simulink model "system_simulation_FC"  (R2025b)
settings: Solver=FixedStepAuto  StartTime=0.0  StopTime=12  FixedStep=Ts/10  RelTol=1e-3
model workspace (MAT data in the model file):
  aprbs_seed = 10
  u_hover = [0.385; 0.385; 0.385; 0.385]
values from neighbouring files (symbols this model uses):
  horizon_N = 20    [main_simulation.m]    (also in random_init.m)
  Ts = 0.05    [generate_commande_preview.m]    (also in random_init.m)
libraries: slpidlib x4
settings Model: Creator=Max  LastModifiedBy=cs_fondation
settings SolverCC: AlgebraicLoopSolver=TrustRegion
settings DebuggingCC: UnconnectedInputMsg=warning  UnconnectedOutputMsg=warning  UnconnectedLineMsg=warning
settings ModelReferenceCC: EnableRefExpFcnMdlSchedulingChecks=on
settings RTWCC: GPUComputeCapability=3.5

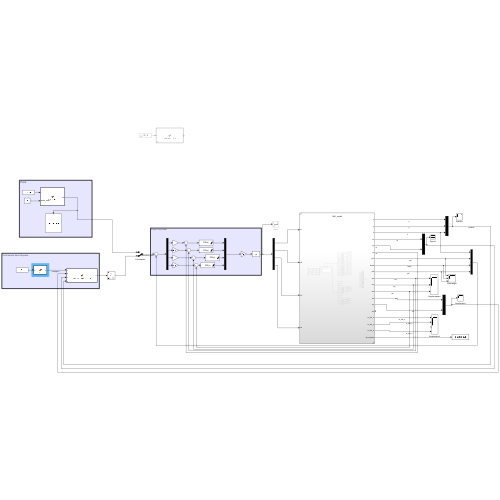
[thumbnail: Simulink's stored preview of the top-level diagram]
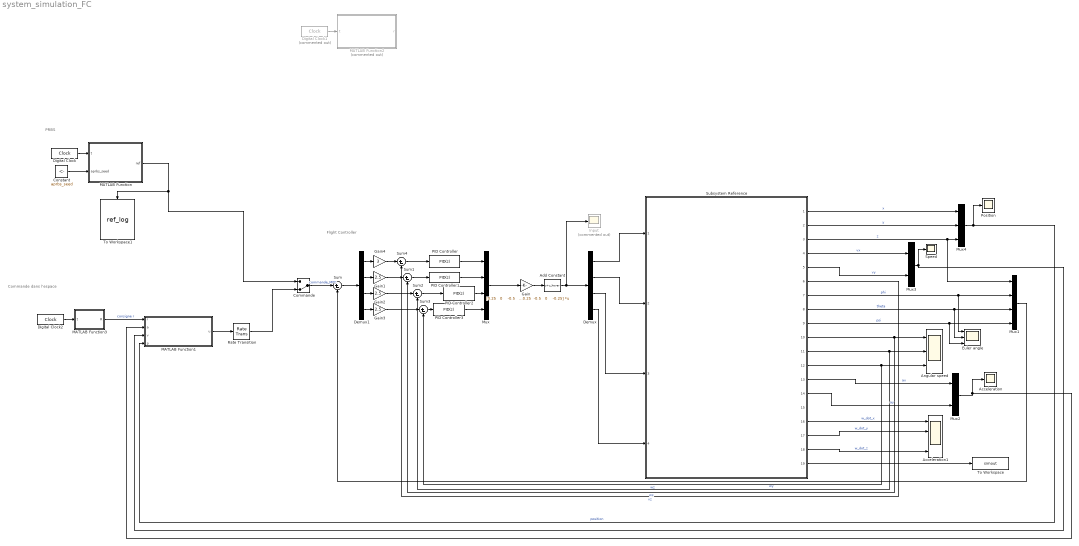
== system system_simulation_FC ==
  note: Commande dans l'espace
  note: Flight Controller
  note: PRBS
  Acceleration : Scope
      settings: ActiveDisplayYMinimum=-12.148465350315172  ActiveDisplayYMaximum=11.235939995916615
  Acceleration1 : Scope  NumInputPorts=4
      settings: ActiveDisplayYMinimum=-40.918121722117149  ActiveDisplayYMaximum=44.001627281329164  DataLoggingVariableName=ScopeData2
  Add Constant : Bias  Bias=u_hover  SaturateOnIntegerOverflow=off
  Angular speed : Scope  NumInputPorts=3
      settings: ActiveDisplayYMinimum=-1  ActiveDisplayYMaximum=1  DataLoggingVariableName=ScopeData3
  Commande : ManualSwitch  CurrentSetting=0
  Constant : Constant  Value=aprbs_seed
  Demux : Demux
  Demux1 : Demux
  Digital Clock : DigitalClock  SampleTime=Ts
  Digital Clock1 : DigitalClock  Commented=on  SampleTime=Ts
  Digital Clock2 : DigitalClock  SampleTime=Ts
  Euler angle : Scope  NumInputPorts=3
      settings: ActiveDisplayYMinimum=-0.25591734670833521  ActiveDisplayYMaximum=0.42163771962698082  DataLoggingVariableName=ScopeData4
  Gain : Gain  Gain=|  Multiplication=Matrix(K*u)
      | [0.25   0    -0.5   0.25;
      |  0.25   0.5   0    -0.25;
      |  0.25   0     0.5   0.25;
      |  0.25  -0.5   0    -0.25]
  Gain1 : Gain  Gain=2.5
  Gain2 : Gain  Gain=2.5
  Gain3 : Gain  Gain=2.5
  Gain4 : Gain  Gain=3
  Input : Scope  Commented=on
      settings: ActiveDisplayYMinimum=-1.25  ActiveDisplayYMaximum=1.25  DataLoggingVariableName=ScopeData5
  MATLAB Function : MATLAB Function  TreatAsAtomicUnit=on
  MATLAB Function1 : MATLAB Function  TreatAsAtomicUnit=on
  MATLAB Function2 : MATLAB Function  Commented=on  TreatAsAtomicUnit=on
  MATLAB Function3 : MATLAB Function  TreatAsAtomicUnit=on
  Mux : Mux
  Mux1 : Mux
  Mux2 : Mux  Inputs=2
  Mux3 : Mux  Inputs=2
  Mux4 : Mux  Inputs=3
  PID Controller : slpidlib/PID Controller  Controller=PID  Form=Parallel  TimeDomain=Discrete-time  UseExternalTs=off  SampleTime=0.005  IntegratorMethod=Forward Euler  FilterMethod=Forward Euler  ControllerParametersSource=internal  P=2.08  I=0.2  UseKiTs=off  D=0.42  UseExternalDerivativeSource=off  N=100  UseFilter=on  TunerSelectOption=Transfer Function Based (PID Tuner App)  InitialConditionSource=internal  InitialConditionForIntegrator=0  InitialConditionForFilter=0  DifferentiatorICPrevScaledInput=0  ExternalReset=none  TrackingMode=off  Kt=1  LimitOutput=on  SatLimitsSource=internal  UpperSaturationLimit=4*(1 - max(u_hover))  LowerSaturationLimit=-4*min(u_hover)  LinearizeAsGain=off  AntiWindupMode=clamping  Kb=1  LimitIntegrator=off  UpperIntegratorSaturationLimit=inf  LowerIntegratorSaturationLimit=-inf  POutMin=[]  POutMax=[]  IOutMin=[]  IOutMax=[]  DOutMin=[]  DOutMax=[]  NOutMin=[]  NOutMax=[]  SumOutMin=[]  SumOutMax=[]  SaturationOutMin=[]  SaturationOutMax=[]  PParamMin=[]  PParamMax=[]  IParamMin=[]  IParamMax=[]  DParamMin=[]  DParamMax=[]  NParamMin=[]  NParamMax=[]  KbParamMin=[]  KbParamMax=[]  KtParamMin=[]  KtParamMax=[]  KbOutMin=[]  KbOutMax=[]  KtOutMin=[]  KtOutMax=[]  IntegratorOutMin=[]  IntegratorOutMax=[]  FilterOutMin=[]  FilterOutMax=[]  SumI1OutMin=[]  SumI1OutMax=[]  SumI2OutMin=[]  SumI2OutMax=[]  SumI3OutMin=[]  SumI3OutMax=[]  SumI4OutMin=[]  SumI4OutMax=[]  SumDOutMin=[]  SumDOutMax=[]  DifferentiatorOutMin=[]  DifferentiatorOutMax=[]  FilterDiffOutCoefMin=[]  FilterDiffOutCoefMax=[]  ReciprocalOutMin=[]  ReciprocalOutMax=[]  SumDenOutMin=[]  SumDenOutMax=[]  SumNumOutMin=[]  SumNumOutMax=[]  DivideOutMin=[]  DivideOutMax=[]  UdiffTsProdOutMin=[]  UdiffTsProdOutMax=[]  NTsProdOutMin=[]  NTsProdOutMax=[]  UintegralTsProdOutMin=[]  UintegralTsProdOutMax=[]  UngainTsProdOutMin=[]  UngainTsProdOutMax=[]  ClampingZeroOutDataTypeStr=Inherit: Inherit via back propagation  ClampingZeroOutMin=[]  ClampingZeroOutMax=[]  FilterDenConstantOutDataTypeStr=Inherit: Inherit via back propagation  FilterDenConstantOutMin=[]  FilterDenConstantOutMax=[]  PCopyOutDataTypeStr=Inherit: Inherit via back propagation  PCopyOutMin=[]  PCopyOutMax=[]  NCopyOutDataTypeStr=Inherit: Inherit via back propagation  NCopyOutMin=[]  NCopyOutMax=[]  IntegratorContinuousStateAttributes=''  IntegratorStateMustResolveToSignalObject=off  IntegratorRTWStateStorageClass=Auto  FilterContinuousStateAttributes=''  FilterStateMustResolveToSignalObject=off  FilterRTWStateStorageClass=Auto  ParallelPVariant=InternalParameters  IdealPVariant=Disabled  IVariant=InternalParameters  DVariant=InternalParameters  IntegratorVariant=Discrete  SatVariant=Enabled  AWVariant=DiscClampingParallel  PCopyVariant=Disabled  TRVariant=Disabled  FdbkBlocksVariant=Forward  IdealPFdbkVariant=Disabled  SatFdbkVariant=Disabled  DerivativeFilterVariant=ForwardEulerFilter  NVariant=InternalParameters  NCopyVariant=Disabled  FilterICVariant=InternalICsFilter  IntegratorICVariant=InternalICs  ExternalResetVariant=Disabled  TRSumVariant=Passthrough  SumFdbkVariant=Disabled  SumVariant=Sum_PID  TsampFilterVariant=InternalTs  TsampNgainVariant=Passthrough  TsampIntegralVariant=Disabled_SignalSpec  ExternalSaturationOutDataTypeStr=Inherit: Same as second input  DerivativeSourceVariant=ErrorSignal  PreIntVariant=InternalPreInt
  PID Controller1 : slpidlib/PID Controller  Controller=PID  Form=Parallel  TimeDomain=Discrete-time  UseExternalTs=off  SampleTime=0.005  IntegratorMethod=Forward Euler  FilterMethod=Forward Euler  ControllerParametersSource=internal  P=0.125  I=0.05  UseKiTs=off  D=0.025  UseExternalDerivativeSource=off  N=100  UseFilter=on  TunerSelectOption=Transfer Function Based (PID Tuner App)  InitialConditionSource=internal  InitialConditionForIntegrator=0  InitialConditionForFilter=0  DifferentiatorICPrevScaledInput=0  ExternalReset=none  TrackingMode=off  Kt=1  LimitOutput=on  SatLimitsSource=internal  UpperSaturationLimit=2*min([u_hover(:); 1 - u_hover(:)])  LowerSaturationLimit=-2*min([u_hover(:); 1 - u_hover(:)])  LinearizeAsGain=on  AntiWindupMode=clamping  Kb=1  LimitIntegrator=off  UpperIntegratorSaturationLimit=inf  LowerIntegratorSaturationLimit=-inf  POutMin=[]  POutMax=[]  IOutMin=[]  IOutMax=[]  DOutMin=[]  DOutMax=[]  NOutMin=[]  NOutMax=[]  SumOutMin=[]  SumOutMax=[]  SaturationOutMin=[]  SaturationOutMax=[]  PParamMin=[]  PParamMax=[]  IParamMin=[]  IParamMax=[]  DParamMin=[]  DParamMax=[]  NParamMin=[]  NParamMax=[]  KbParamMin=[]  KbParamMax=[]  KtParamMin=[]  KtParamMax=[]  KbOutMin=[]  KbOutMax=[]  KtOutMin=[]  KtOutMax=[]  IntegratorOutMin=[]  IntegratorOutMax=[]  FilterOutMin=[]  FilterOutMax=[]  SumI1OutMin=[]  SumI1OutMax=[]  SumI2OutMin=[]  SumI2OutMax=[]  SumI3OutMin=[]  SumI3OutMax=[]  SumI4OutMin=[]  SumI4OutMax=[]  SumDOutMin=[]  SumDOutMax=[]  DifferentiatorOutMin=[]  DifferentiatorOutMax=[]  FilterDiffOutCoefMin=[]  FilterDiffOutCoefMax=[]  ReciprocalOutMin=[]  ReciprocalOutMax=[]  SumDenOutMin=[]  SumDenOutMax=[]  SumNumOutMin=[]  SumNumOutMax=[]  DivideOutMin=[]  DivideOutMax=[]  UdiffTsProdOutMin=[]  UdiffTsProdOutMax=[]  NTsProdOutMin=[]  NTsProdOutMax=[]  UintegralTsProdOutMin=[]  UintegralTsProdOutMax=[]  UngainTsProdOutMin=[]  UngainTsProdOutMax=[]  ClampingZeroOutDataTypeStr=Inherit: Inherit via back propagation  ClampingZeroOutMin=[]  ClampingZeroOutMax=[]  FilterDenConstantOutDataTypeStr=Inherit: Inherit via back propagation  FilterDenConstantOutMin=[]  FilterDenConstantOutMax=[]  PCopyOutDataTypeStr=Inherit: Inherit via back propagation  PCopyOutMin=[]  PCopyOutMax=[]  NCopyOutDataTypeStr=Inherit: Inherit via back propagation  NCopyOutMin=[]  NCopyOutMax=[]  IntegratorContinuousStateAttributes=''  IntegratorStateMustResolveToSignalObject=off  IntegratorRTWStateStorageClass=Auto  FilterContinuousStateAttributes=''  FilterStateMustResolveToSignalObject=off  FilterRTWStateStorageClass=Auto  ParallelPVariant=InternalParameters  IdealPVariant=Disabled  IVariant=InternalParameters  DVariant=InternalParameters  IntegratorVariant=Discrete  SatVariant=Enabled  AWVariant=DiscClampingParallel  PCopyVariant=Disabled  TRVariant=Disabled  FdbkBlocksVariant=Forward  IdealPFdbkVariant=Disabled  SatFdbkVariant=Disabled  DerivativeFilterVariant=ForwardEulerFilter  NVariant=InternalParameters  NCopyVariant=Disabled  FilterICVariant=InternalICsFilter  IntegratorICVariant=InternalICs  ExternalResetVariant=Disabled  TRSumVariant=Passthrough  SumFdbkVariant=Disabled  SumVariant=Sum_PID  TsampFilterVariant=InternalTs  TsampNgainVariant=Passthrough  TsampIntegralVariant=Disabled_SignalSpec  ExternalSaturationOutDataTypeStr=Inherit: Same as second input  DerivativeSourceVariant=ErrorSignal  PreIntVariant=InternalPreInt
  PID Controller2 : slpidlib/PID Controller  Controller=PID  Form=Parallel  TimeDomain=Discrete-time  UseExternalTs=off  SampleTime=0.005  IntegratorMethod=Forward Euler  FilterMethod=Forward Euler  ControllerParametersSource=internal  P=0.125  I=0.05  UseKiTs=off  D=0.025  UseExternalDerivativeSource=off  N=100  UseFilter=on  TunerSelectOption=Transfer Function Based (PID Tuner App)  InitialConditionSource=internal  InitialConditionForIntegrator=0  InitialConditionForFilter=0  DifferentiatorICPrevScaledInput=0  ExternalReset=none  TrackingMode=off  Kt=1  LimitOutput=on  SatLimitsSource=internal  UpperSaturationLimit=2*min([u_hover(:); 1 - u_hover(:)])  LowerSaturationLimit=-2*min([u_hover(:); 1 - u_hover(:)])  LinearizeAsGain=on  AntiWindupMode=clamping  Kb=1  LimitIntegrator=off  UpperIntegratorSaturationLimit=inf  LowerIntegratorSaturationLimit=-inf  POutMin=[]  POutMax=[]  IOutMin=[]  IOutMax=[]  DOutMin=[]  DOutMax=[]  NOutMin=[]  NOutMax=[]  SumOutMin=[]  SumOutMax=[]  SaturationOutMin=[]  SaturationOutMax=[]  PParamMin=[]  PParamMax=[]  IParamMin=[]  IParamMax=[]  DParamMin=[]  DParamMax=[]  NParamMin=[]  NParamMax=[]  KbParamMin=[]  KbParamMax=[]  KtParamMin=[]  KtParamMax=[]  KbOutMin=[]  KbOutMax=[]  KtOutMin=[]  KtOutMax=[]  IntegratorOutMin=[]  IntegratorOutMax=[]  FilterOutMin=[]  FilterOutMax=[]  SumI1OutMin=[]  SumI1OutMax=[]  SumI2OutMin=[]  SumI2OutMax=[]  SumI3OutMin=[]  SumI3OutMax=[]  SumI4OutMin=[]  SumI4OutMax=[]  SumDOutMin=[]  SumDOutMax=[]  DifferentiatorOutMin=[]  DifferentiatorOutMax=[]  FilterDiffOutCoefMin=[]  FilterDiffOutCoefMax=[]  ReciprocalOutMin=[]  ReciprocalOutMax=[]  SumDenOutMin=[]  SumDenOutMax=[]  SumNumOutMin=[]  SumNumOutMax=[]  DivideOutMin=[]  DivideOutMax=[]  UdiffTsProdOutMin=[]  UdiffTsProdOutMax=[]  NTsProdOutMin=[]  NTsProdOutMax=[]  UintegralTsProdOutMin=[]  UintegralTsProdOutMax=[]  UngainTsProdOutMin=[]  UngainTsProdOutMax=[]  ClampingZeroOutDataTypeStr=Inherit: Inherit via back propagation  ClampingZeroOutMin=[]  ClampingZeroOutMax=[]  FilterDenConstantOutDataTypeStr=Inherit: Inherit via back propagation  FilterDenConstantOutMin=[]  FilterDenConstantOutMax=[]  PCopyOutDataTypeStr=Inherit: Inherit via back propagation  PCopyOutMin=[]  PCopyOutMax=[]  NCopyOutDataTypeStr=Inherit: Inherit via back propagation  NCopyOutMin=[]  NCopyOutMax=[]  IntegratorContinuousStateAttributes=''  IntegratorStateMustResolveToSignalObject=off  IntegratorRTWStateStorageClass=Auto  FilterContinuousStateAttributes=''  FilterStateMustResolveToSignalObject=off  FilterRTWStateStorageClass=Auto  ParallelPVariant=InternalParameters  IdealPVariant=Disabled  IVariant=InternalParameters  DVariant=InternalParameters  IntegratorVariant=Discrete  SatVariant=Enabled  AWVariant=DiscClampingParallel  PCopyVariant=Disabled  TRVariant=Disabled  FdbkBlocksVariant=Forward  IdealPFdbkVariant=Disabled  SatFdbkVariant=Disabled  DerivativeFilterVariant=ForwardEulerFilter  NVariant=InternalParameters  NCopyVariant=Disabled  FilterICVariant=InternalICsFilter  IntegratorICVariant=InternalICs  ExternalResetVariant=Disabled  TRSumVariant=Passthrough  SumFdbkVariant=Disabled  SumVariant=Sum_PID  TsampFilterVariant=InternalTs  TsampNgainVariant=Passthrough  TsampIntegralVariant=Disabled_SignalSpec  ExternalSaturationOutDataTypeStr=Inherit: Same as second input  DerivativeSourceVariant=ErrorSignal  PreIntVariant=InternalPreInt
  PID Controller3 : slpidlib/PID Controller  Controller=PID  Form=Parallel  TimeDomain=Discrete-time  UseExternalTs=off  SampleTime=0.005  IntegratorMethod=Forward Euler  FilterMethod=Forward Euler  ControllerParametersSource=internal  P=0.23  I=0.093  UseKiTs=off  D=0.047  UseExternalDerivativeSource=off  N=100  UseFilter=on  TunerSelectOption=Transfer Function Based (PID Tuner App)  InitialConditionSource=internal  InitialConditionForIntegrator=0  InitialConditionForFilter=0  DifferentiatorICPrevScaledInput=0  ExternalReset=none  TrackingMode=off  Kt=1  LimitOutput=on  SatLimitsSource=internal  UpperSaturationLimit=2*min([u_hover(:); 1 - u_hover(:)])  LowerSaturationLimit=-2*min([u_hover(:); 1 - u_hover(:)])  LinearizeAsGain=on  AntiWindupMode=none  Kb=1  LimitIntegrator=off  UpperIntegratorSaturationLimit=inf  LowerIntegratorSaturationLimit=-inf  POutMin=[]  POutMax=[]  IOutMin=[]  IOutMax=[]  DOutMin=[]  DOutMax=[]  NOutMin=[]  NOutMax=[]  SumOutMin=[]  SumOutMax=[]  SaturationOutMin=[]  SaturationOutMax=[]  PParamMin=[]  PParamMax=[]  IParamMin=[]  IParamMax=[]  DParamMin=[]  DParamMax=[]  NParamMin=[]  NParamMax=[]  KbParamMin=[]  KbParamMax=[]  KtParamMin=[]  KtParamMax=[]  KbOutMin=[]  KbOutMax=[]  KtOutMin=[]  KtOutMax=[]  IntegratorOutMin=[]  IntegratorOutMax=[]  FilterOutMin=[]  FilterOutMax=[]  SumI1OutMin=[]  SumI1OutMax=[]  SumI2OutMin=[]  SumI2OutMax=[]  SumI3OutMin=[]  SumI3OutMax=[]  SumI4OutMin=[]  SumI4OutMax=[]  SumDOutMin=[]  SumDOutMax=[]  DifferentiatorOutMin=[]  DifferentiatorOutMax=[]  FilterDiffOutCoefMin=[]  FilterDiffOutCoefMax=[]  ReciprocalOutMin=[]  ReciprocalOutMax=[]  SumDenOutMin=[]  SumDenOutMax=[]  SumNumOutMin=[]  SumNumOutMax=[]  DivideOutMin=[]  DivideOutMax=[]  UdiffTsProdOutMin=[]  UdiffTsProdOutMax=[]  NTsProdOutMin=[]  NTsProdOutMax=[]  UintegralTsProdOutMin=[]  UintegralTsProdOutMax=[]  UngainTsProdOutMin=[]  UngainTsProdOutMax=[]  ClampingZeroOutDataTypeStr=Inherit: Inherit via back propagation  ClampingZeroOutMin=[]  ClampingZeroOutMax=[]  FilterDenConstantOutDataTypeStr=Inherit: Inherit via back propagation  FilterDenConstantOutMin=[]  FilterDenConstantOutMax=[]  PCopyOutDataTypeStr=Inherit: Inherit via back propagation  PCopyOutMin=[]  PCopyOutMax=[]  NCopyOutDataTypeStr=Inherit: Inherit via back propagation  NCopyOutMin=[]  NCopyOutMax=[]  IntegratorContinuousStateAttributes=''  IntegratorStateMustResolveToSignalObject=off  IntegratorRTWStateStorageClass=Auto  FilterContinuousStateAttributes=''  FilterStateMustResolveToSignalObject=off  FilterRTWStateStorageClass=Auto  ParallelPVariant=InternalParameters  IdealPVariant=Disabled  IVariant=InternalParameters  DVariant=InternalParameters  IntegratorVariant=Discrete  SatVariant=Enabled  AWVariant=Passthrough  PCopyVariant=Disabled  TRVariant=Disabled  FdbkBlocksVariant=Forward  IdealPFdbkVariant=Disabled  SatFdbkVariant=Disabled  DerivativeFilterVariant=ForwardEulerFilter  NVariant=InternalParameters  NCopyVariant=Disabled  FilterICVariant=InternalICsFilter  IntegratorICVariant=InternalICs  ExternalResetVariant=Disabled  TRSumVariant=Passthrough  SumFdbkVariant=Disabled  SumVariant=Sum_PID  TsampFilterVariant=InternalTs  TsampNgainVariant=Passthrough  TsampIntegralVariant=Disabled_SignalSpec  ExternalSaturationOutDataTypeStr=Inherit: Same as second input  DerivativeSourceVariant=ErrorSignal  PreIntVariant=InternalPreInt
  Position : Scope
      settings: ActiveDisplayYMinimum=-0.2899549745941804  ActiveDisplayYMaximum=1.2517165940077446  DataLoggingVariableName=ScopeData6
  Rate Transition : RateTransition  OutPortSampleTime=Ts/10
  Speed : Scope
      settings: ActiveDisplayYMinimum=-29.1666816614834  ActiveDisplayYMaximum=149.08188384676708
  Subsystem Reference : Subsystem  ReferencedSubsystem=UAV_model
  Sum{,1..4} (5 alike) : Sum  Inputs=|+-
  To Workspace : ToWorkspace  VariableName=simout  SaveFormat=Structure With Time  SampleTime=Ts
  To Workspace1 : ToWorkspace  VariableName=ref_log  SaveFormat=Structure With Time  SampleTime=Ts
  wires:
  Subsystem Reference/18 -> Acceleration1/4  "w_dot_z"
  Subsystem Reference/12 -> Angular speed/3, Sum3/2  "wz"
  Subsystem Reference/17 -> Acceleration1/2  "w_dot_y"
  Subsystem Reference/9 -> Mux1/4, Euler angle/3  "psi"
  Subsystem Reference/8 -> Mux1/3, Euler angle/2  "theta"
  Subsystem Reference/14 -> Mux2/2  "ay"
  Subsystem Reference/10 -> Angular speed/1, Sum1/2  "wx"
  Subsystem Reference/2 -> Mux4/2  "y"
  Subsystem Reference/13 -> Mux2/1  "ax"
  Subsystem Reference/16 -> Acceleration1/1  "w_dot_x"
  Subsystem Reference/7 -> Mux1/2, Euler angle/1  "phi"
  Subsystem Reference/19 -> To Workspace/1
  Subsystem Reference/1 -> Mux4/1  "x"
  Subsystem Reference/6 -> Sum4/2  "vz"
  Subsystem Reference/4 -> Mux3/1  "vx"
  Subsystem Reference/3 -> Mux4/3, Mux1/1  "z"
  Subsystem Reference/11 -> Angular speed/2, Sum2/2  "wy"
  PID Controller/1 -> Mux/1
  PID Controller2/1 -> Mux/3
  Mux/1 -> Gain/1
  Demux/1 -> Subsystem Reference/1
  Demux/2 -> Subsystem Reference/2
  Demux/3 -> Subsystem Reference/3
  Demux/4 -> Subsystem Reference/4
  Gain/1 -> Add Constant/1
  Demux1/2 -> Gain1/1
  Add Constant/1 -> Demux/1, Input/1
  Mux1/1 -> Sum/2
  PID Controller1/1 -> Mux/2
  Sum/1 -> Demux1/1
  Gain1/1 -> Sum1/1
  Sum1/1 -> PID Controller1/1
  Sum2/1 -> PID Controller2/1
  Gain2/1 -> Sum2/1
  Demux1/3 -> Gain2/1
  Demux1/4 -> Gain3/1
  Gain3/1 -> Sum3/1
  Sum3/1 -> PID Controller3/1
  PID Controller3/1 -> Mux/4
  Demux1/1 -> Gain4/1
  Gain4/1 -> Sum4/1
  Sum4/1 -> PID Controller/1
  Digital Clock/1 -> MATLAB Function/1(t)
  MATLAB Function/1(ref) -> Commande/1, To Workspace1/1
  Constant/1 -> MATLAB Function/2(aprbs_seed)
  Commande/1 -> Sum/1  "commande_MPC"
  Mux2/1 -> Acceleration/1, MATLAB Function1/2(a)
  Mux3/1 -> MATLAB Function1/3(v), Speed/1
  Mux4/1 -> Position/1, MATLAB Function1/4(p)  "position"
  MATLAB Function1/1(u) -> Rate Transition/1
  Rate Transition/1 -> Commande/2
  MATLAB Function3/1(R) -> MATLAB Function1/1(r)  "consigne r"
  Digital Clock1/1 -> MATLAB Function2/1(t)
  Subsystem Reference/5 -> Mux3/2  "vy"
  Digital Clock2/1 -> MATLAB Function3/1(t)

== matlab function system_simulation_FC/MATLAB Function ==
  settings: updateMethod=DISCRETE
  data: ref output; t input; aprbs_seed input
function ref = aprbs_ref(t, aprbs_seed)
% Consignes APRBS : ref = [z_ref; phi_ref; theta_ref; psi_ref]
% Paliers de durée aléatoire entre Tmin et Tmax (tirage log-uniforme)

T_warm = 3;                        % [s] démarrage moteurs : stationnaire à 1 m
dt_ref = 0.05;                     % [s] grille des consignes (20 Hz)
Tmin = [0.5; 0.25; 0.25; 0.4];     % [s] durée min d'un palier : z, phi, theta, psi
Tmax = [8.0; 5.0;  5.0;  6.0];     % [s] durée max d'un palier
lo   = [-1; -0.3; -0.3; -0.5];    % niveaux min (m, rad, rad, rad)
hi   = [2.5;  0.3;  0.3;  0.5];    % niveaux max
NMAX = 1000;                       % paliers pré-calculés par canal (>= 250 s couverts)

persistent tchg lev kcur
if isempty(tchg)
    rng(aprbs_seed);
    tchg = zeros(NMAX, 4);         % instant de début de chaque palier (après T_warm)
    lev  = zeros(NMAX, 4);         % niveau de chaque palier
    kcur = ones(4, 1);             % palier en cours, par canal
    for c = 1:4
        tc = 0;
        for k = 1:NMAX
            tchg(k, c) = tc;
            lev(k, c)  = lo(c) + (hi(c) - lo(c)) * rand;
            % durée log-uniforme entre Tmin et Tmax, arrondie à la grille 20 Hz
            d  = exp(log(Tmin(c)) + (log(Tmax(c)) - log(Tmin(c))) * rand);
            d  = max(dt_ref, round(d / dt_ref) * dt_ref);
            tc = tc + d;
        end
    end
end

ref = zeros(4, 1);
if t < T_warm
    ref(1) = 1;                    % décollage à 1 m, angles à 0
else
    tau = t - T_warm + 1e-9;       % 1e-9 : évite les erreurs d'arrondi
    for c = 1:4
        while kcur(c) < NMAX && tau >= tchg(kcur(c) + 1, c)
            kcur(c) = kcur(c) + 1;
        end
        ref(c) = lev(kcur(c), c);
    end
end

== matlab function system_simulation_FC/MATLAB Function1 ==
  settings: updateMethod=DISCRETE  sampleTime=Ts
  data: r input; a input; u output; v input; p input
function u = mpc_controller_block(r, a, v, p)
    %#codegen
    persistent controller

    coder.extrinsic('evalin', 'step');

    u = zeros(4, 1);   % [z_ref; phi_ref; theta_ref; psi_ref]

    if isempty(controller)
        controller = evalin('base', 'mpc_system');
    end
    u = step(controller, r, a, v, p);
end

== matlab function system_simulation_FC/MATLAB Function2 ==
  settings: updateMethod=DISCRETE  sampleTime=Ts
  data: t input; r output; horizon_N parameter; Ts parameter
function r = space_command(t, horizon_N, Ts)
    coder.extrinsic('commande_space_step');
    t_future = t + (0:horizon_N-1)' * Ts;
    r_tmp = zeros(horizon_N, 3);
    r_tmp = commande_space_step(t_future);
    r = r_tmp.';
end

== matlab function system_simulation_FC/MATLAB Function3 ==
  data: t input; R output
function R = car_ref(t)
% Bloc MATLAB Function : entrée t depuis un Digital Clock (Sample time = Ts).
% Sortie R (3 x N) : consigne [x; y; z] du drone sur les N pas de l'horizon,
% aux instants t, t+Ts, ..., t+(N-1)*Ts.
%   x, y : position de la voiture (plan z = 0)
%   z    : 0.5 m en suivi, 2 m au passage du pont (reste dans [-1 ; 2.5], le domaine du RNN)
% Toutes les transitions sont en polynôme de degré 5 : vitesse et accélération
% continues, donc des consignes d'angle sans à-coup pour le FC.
% Stop Time conseillé : 38 s.

Ts = 0.05;           % doit être égal au Ts de random_init
N  = 20;             % horizon du MPC
tk = t + (0:N-1)*Ts;

% --- voiture : arrêt jusqu'à 4 s (stabilisation du drone, comme T_warm du dataset),
%     croisière à 1.5 m/s sur une route qui ondule doucement, arrêt à 33 s (x = 36 m)
V  = 1.5;            % vitesse de croisière [m/s]
t0 = 4;  Ta = 5;     % début et durée de l'accélération [s]
t1 = 28; Td = 5;     % début et durée du freinage [s]
A  = 1;  L = 20;     % ondulation en y : amplitude [m], longueur d'onde [m]
s  = V*(Ta*g((tk - t0)/Ta) - Td*g((tk - t1)/Td));
x  = s;
y  = A*sin(2*pi*s/L);

% --- pont entre x = 24 et 27 m (tablier entre 1.4 et 1.6 m) :
%     la voiture passe dessous de 22.5 à 24.5 s
xb_in = 24;  xb_out = 27;
z_follow = 0.5;      % altitude de suivi [m]
z_bridge = 2.0;      % altitude au-dessus du pont [m], < 2.5 (max vu par le RNN)
T_ramp   = 3;        % durée de la montée et de la descente [s]
t_in  = t0 + Ta/2 + xb_in/V;     % entrée sous le pont (22.5 s)
t_out = t0 + Ta/2 + xb_out/V;    % sortie (24.5 s)
z = z_follow + (z_bridge - z_follow) * ...
    (sstep((tk - (t_in - T_ramp))/T_ramp) - sstep((tk - t_out)/T_ramp));

R = [x; y; z];
end

function G = g(tau)
% distance parcourue normalisée pendant une accélération douce (intégrale de sstep)
tc = min(max(tau, 0), 1);
G  = tc.^6 - 3*tc.^5 + 2.5*tc.^4 + max(tau - 1, 0);
end

function S = sstep(tau)
% passage doux de 0 à 1, vitesse et accélération nulles aux deux bouts
tc = min(max(tau, 0), 1);
S  = 6*tc.^5 - 15*tc.^4 + 10*tc.^3;
end
